simulink model "UAM_Hexa_PD_Obs_QGround"  (R2026a)
settings: Solver=ode4  StopTime=tf  FixedStep=0.01  EnableMultiTasking=on
values from neighbouring files (symbols this model uses):
  ArmConstants = struct('l1_dim', l1_dim,                        'l2_dim', l2_dim,                        'Hexa_to_joint_L', L,                        'Mass1', ml1,                        'Mass2', ml2,                        'Inertia1', Hl1,                        'Inertia2', Hl2,                        'MC1', c1,                        'MC2', c2,                        'Servos', Servos)    [init_model.m]    (also in init_var.m)
  HexaConstants = struct('Mass', mb,                         'Inertia', J ,                         'allo', allo,                          'invallo', invallo,                         'kT', kT)    [init_model.m]    (also in init_var.m)
  Observer = struct('E1', E1 ,     'E2', E2 ,     'E3', E3 ,     'E4', E4 ,     'MU1', MU1 ,     'MU2', MU2 ,     'MU3', MU3 ,     'alpha', alpha ,     'beta', beta)    [init_model.m]    (also in init_var.m)
libraries: px4Utilslib x189
(part 2 of 2)

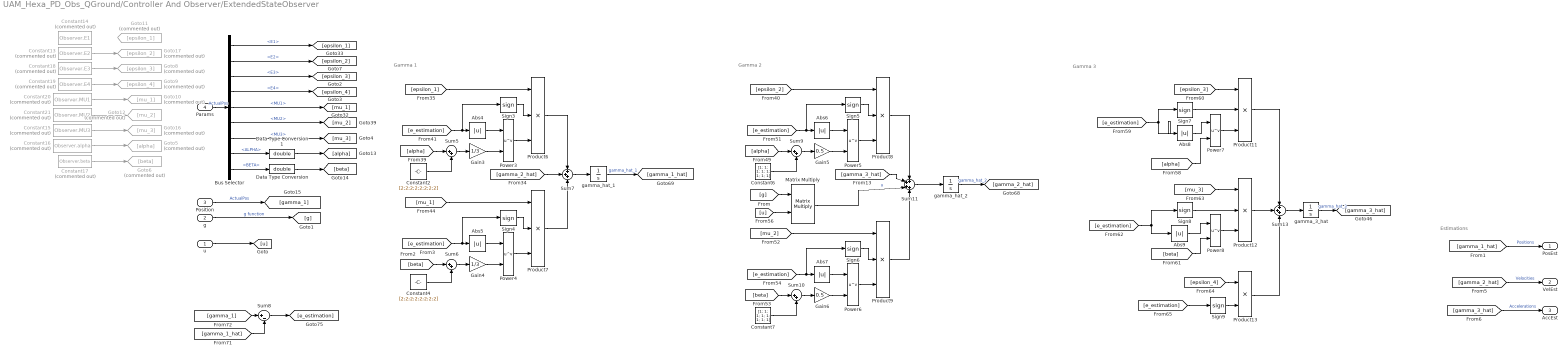
== system UAM_Hexa_PD_Obs_QGround/Controller And Observer/ExtendedStateObserver ==
  note: Estimations
  note: Gamma 3
  note: Gamma 2
  note: Gamma 1
  u : Inport  SampleTime=0.01
  g : Inport  Port=2  SampleTime=0.01
  Position : Inport  Port=3  SampleTime=0.01
  Params : Inport  Port=4  SampleTime=0.01
  Abs{4..9} (6 alike) : Abs  SaturateOnIntegerOverflow=off
  Bus Selector : BusSelector  OutputSignals=E1,E2,E3,E4,MU1,MU2,MU3,ALPHA,BETA
  Constant13 : Constant  Commented=on  Value=Observer.E2
  Constant14 : Constant  Commented=on  Value=Observer.E1
  Constant15 : Constant  Commented=on  Value=Observer.MU3
  Constant16 : Constant  Commented=on  Value=Observer.alpha
  Constant17 : Constant  Commented=on  Value=Observer.beta
  Constant18 : Constant  Commented=on  Value=Observer.E3
  Constant19 : Constant  Commented=on  Value=Observer.E4
  Constant2 : Constant  Value=[2;2;2;2;2;2;2;2]
  Constant20 : Constant  Commented=on  Value=Observer.MU1
  Constant21 : Constant  Commented=on  Value=Observer.MU2
  Constant4 : Constant  Value=[2;2;2;2;2;2;2;2]
  Constant6 : Constant  Value=[1; 1; 1; 1; 1; 1; 1; 1]
  Constant7 : Constant  Value=[1; 1; 1; 1; 1; 1; 1; 1]
  Data Type Conversion : DataTypeConversion  OutDataTypeStr=double  SaturateOnIntegerOverflow=off  RndMeth=Floor
  Data Type Conversion1 : DataTypeConversion  OutDataTypeStr=double  SaturateOnIntegerOverflow=off  RndMeth=Floor
  Gain3 : Gain  Gain=1/3
  Gain4 : Gain  Gain=1/3
  Gain5 : Gain  Gain=0.5
  Gain6 : Gain  Gain=0.5
  Goto10 : Goto  Commented=on  GotoTag=mu_1
  Goto11 : Goto  Commented=on  GotoTag=epsilon_1
  Goto12 : Goto  Commented=on  GotoTag=mu_2
  Goto16 : Goto  Commented=on  GotoTag=mu_3
  Goto17 : Goto  Commented=on  GotoTag=epsilon_2
  Goto5 : Goto  Commented=on  GotoTag=alpha
  Goto6 : Goto  Commented=on  GotoTag=beta
  Goto8 : Goto  Commented=on  GotoTag=epsilon_3
  Goto9 : Goto  Commented=on  GotoTag=epsilon_4
  Matrix Multiply : Product  Multiplication=Matrix(*)
  Power{3..8} (6 alike) : Math  Operator=pow
  Product{6..9,11..12} (6 alike) : Product  Inputs=3
  Product13 : Product
  Sign{3..9} (7 alike) : Signum
  Sum{5..6,9..10} (4 alike) : Sum  Inputs=|++
  Sum11 : Sum  Inputs=++++
  Sum13 : Sum  Inputs=+++
  Sum7 : Sum  Inputs=+++
  Sum8 : Sum  Inputs=|+-
  gamma_3_hat : Integrator  InitialCondition=[0; 0; -9.81; 0; 0; 0; 0; 0]
  gamma_hat_1 : Integrator  InitialCondition=[0; 0; 0.24; 0; 0; 0; 0; 0]
  gamma_hat_2 : Integrator  InitialCondition=zeros(8,1)
  PosEst : Outport  SampleTime=0.01
  VelEst : Outport  Port=2  SampleTime=0.01
  AccEst : Outport  Port=3  SampleTime=0.01
  wires:
  Bus Selector/8 -> Data Type Conversion1/1  "<ALPHA>"
  [beta] -> Sum10/1
  [e_estimation] -> Sign8/1, Abs9/1
  Power7/1 -> Product11/3
  Matrix Multiply/1 -> Sum11/3  "u"
  Bus Selector/9 -> Data Type Conversion/1  "<BETA>"
  [e_estimation] -> Abs8/1, Sign7/1
  [gamma_1_hat] -> PosEst/1  "Positions"
  Power8/1 -> Product12/3
  Constant4/1 -> Sum6/2
  [alpha] -> Sum5/1
  Product6/1 -> Sum7/1
  Abs8/1 -> Power7/1
  Power5/1 -> Product8/3
  [gamma_1] -> Sum8/1
  [e_estimation] -> Sign6/1, Abs7/1
  [epsilon_2] -> Product8/1
  Sum11/1 -> gamma_hat_2/1
  Bus Selector/7 -> [mu_3]  "<MU3>"
  Gain5/1 -> Power5/2
  [e_estimation] -> Sign3/1, Abs4/1
  Abs5/1 -> Power4/1
  Sum13/1 -> gamma_3_hat/1
  Abs7/1 -> Power6/1
  Product9/1 -> Sum11/4
  [epsilon_1] -> Product6/1
  Constant7/1 -> Sum10/2
  [epsilon_3] -> Product11/1
  Sum9/1 -> Gain5/1
  Sum6/1 -> Gain4/1
  [e_estimation] -> Sign5/1, Abs6/1
  u/1 -> [u]
  [mu_3] -> Product12/1
  Sign6/1 -> Product9/2
  Sum7/1 -> gamma_hat_1/1
  Sign8/1 -> Product12/2
  [alpha] -> Power7/2
  [epsilon_4] -> Product13/1
  [gamma_3_hat] -> Sum11/2
  [mu_1] -> Product7/1
  Sign3/1 -> Product6/2
  gamma_hat_2/1 -> [gamma_2_hat]  "gamma_hat_2"
  Bus Selector/2 -> [epsilon_2]  "<E2>"
  [mu_2] -> Product9/1
  Product11/1 -> Sum13/1
  [gamma_1_hat] -> Sum8/2
  Sign4/1 -> Product7/2
  Product7/1 -> Sum7/3
  Bus Selector/6 -> [mu_2]  "<MU2>"
  Bus Selector/1 -> [epsilon_1]  "<E1>"
  Constant6/1 -> Sum9/2
  Sign5/1 -> Product8/2
  [beta] -> Power8/2
  Constant2/1 -> Sum5/2
  Gain6/1 -> Power6/2
  Gain3/1 -> Power3/2
  Power6/1 -> Product9/3
  Position/1 -> [gamma_1]  "ActualPos"
  Bus Selector/4 -> [epsilon_4]  "<E4>"
  Product13/1 -> Sum13/3
  gamma_hat_1/1 -> [gamma_1_hat]  "gamma_hat_1"
  Sum5/1 -> Gain3/1
  Power3/1 -> Product6/3
  Power4/1 -> Product7/3
  Sum10/1 -> Gain6/1
  [gamma_2_hat] -> Sum7/2
  Sign7/1 -> Product11/2
  [beta] -> Sum6/1
  [e_estimation] -> Sign4/1, Abs5/1
  [e_estimation] -> Sign9/1
  Product8/1 -> Sum11/1
  Sign9/1 -> Product13/2
  Abs9/1 -> Power8/1
  [alpha] -> Sum9/1
  gamma_3_hat/1 -> [gamma_3_hat]  "gamma_hat_3"
  Sum8/1 -> [e_estimation]
  Gain4/1 -> Power4/2
  Bus Selector/5 -> [mu_1]  "<MU1>"
  Product12/1 -> Sum13/2
  g/1 -> [g]  "g function"
  Abs6/1 -> Power5/1
  Abs4/1 -> Power3/1
  [gamma_3_hat] -> AccEst/1  "Accelerations"
  [gamma_2_hat] -> VelEst/1  "Velocities"
  [g] -> Matrix Multiply/1
  [u] -> Matrix Multiply/2
  Params/1 -> Bus Selector/1  "ActualPos"
  Constant18/1 -> Goto8/1
  Constant20/1 -> Goto10/1
  Constant21/1 -> Goto12/1
  Constant15/1 -> Goto16/1
  Constant19/1 -> Goto9/1
  Constant17/1 -> Goto6/1
  Constant16/1 -> Goto5/1
  Constant13/1 -> Goto17/1
  Bus Selector/3 -> [epsilon_3]  "<E3>"
  Data Type Conversion/1 -> [beta]
  Data Type Conversion1/1 -> [alpha]

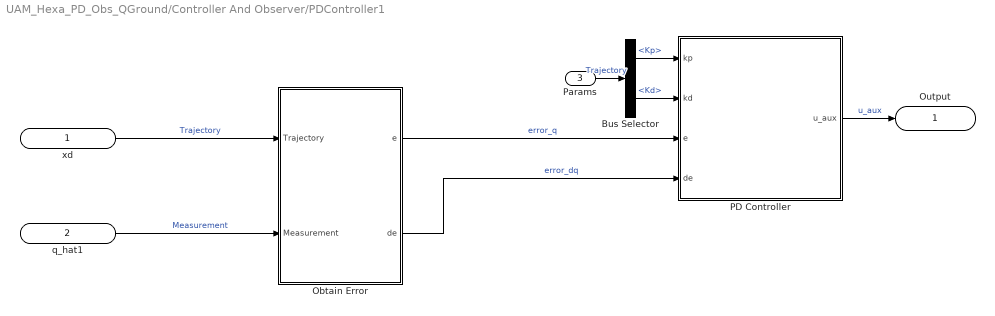
== system UAM_Hexa_PD_Obs_QGround/Controller And Observer/PDController1 ==
  xd : Inport
  q_hat1 : Inport  Port=2
  Params : Inport  Port=3
  Bus Selector : BusSelector  OutputSignals=Kp,Kd
  Obtain Error : Subsystem
  PD Controller : MATLAB Function  TreatAsAtomicUnit=on
  Output : Outport
  wires:
  xd/1 -> Obtain Error/1(Trajectory)  "Trajectory"
  q_hat1/1 -> Obtain Error/2(Measurement)  "Measurement"
  Obtain Error/1(e) -> PD Controller/3(e)  "error_q"
  Obtain Error/2(de) -> PD Controller/4(de)  "error_dq"
  Bus Selector/1 -> PD Controller/1(kp)  "<Kp>"
  Bus Selector/2 -> PD Controller/2(kd)  "<Kd>"
  PD Controller/1(u_aux) -> Output/1  "u_aux"
  Params/1 -> Bus Selector/1  "Trajectory"

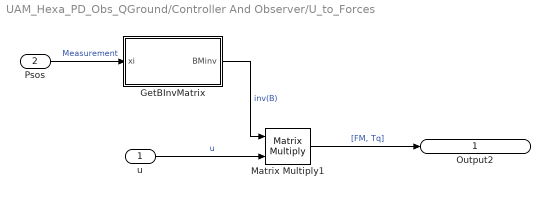
== system UAM_Hexa_PD_Obs_QGround/Controller And Observer/U_to_Forces ==
  u : Inport  SampleTime=0.01
  Psos : Inport  Port=2  SampleTime=0.01
  GetBInvMatrix : MATLAB Function  TreatAsAtomicUnit=on
  Matrix Multiply1 : Product  Multiplication=Matrix(*)
  Output2 : Outport  SampleTime=0.01
  wires:
  Psos/1 -> GetBInvMatrix/1(xi)  "Measurement"
  u/1 -> Matrix Multiply1/2  "u"
  Matrix Multiply1/1 -> Output2/1  "[FM, Tq]"
  GetBInvMatrix/1(BMinv) -> Matrix Multiply1/1  "inv(B)"

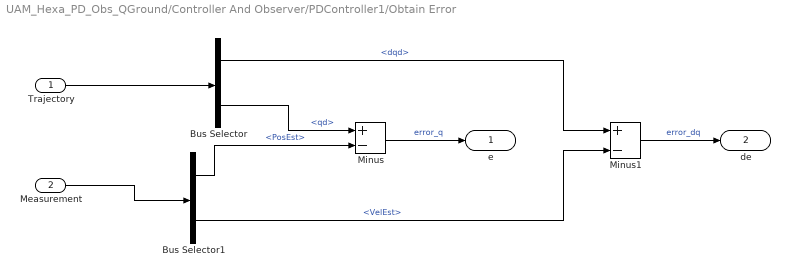
== system UAM_Hexa_PD_Obs_QGround/Controller And Observer/PDController1/Obtain Error ==
  Trajectory : Inport
  Measurement : Inport  Port=2
  Bus Selector : BusSelector  OutputSignals=dqd,qd
  Bus Selector1 : BusSelector  OutputSignals=PosEst,VelEst
  Minus : Sum  Inputs=+-
  Minus1 : Sum  Inputs=+-
  e : Outport
  de : Outport  Port=2
  wires:
  Bus Selector1/1 -> Minus/2  "<PosEst>"
  Bus Selector1/2 -> Minus1/2  "<VelEst>"
  Measurement/1 -> Bus Selector1/1
  Trajectory/1 -> Bus Selector/1
  Bus Selector/1 -> Minus1/1  "<dqd>"
  Bus Selector/2 -> Minus/1  "<qd>"
  Minus/1 -> e/1  "error_q"
  Minus1/1 -> de/1  "error_dq"

== matlab function UAM_Hexa_PD_Obs_QGround/Controller And Observer/PDController1/PD Controller ==
  data: kp input; kd input; u_aux output; e input; de input
function u_aux = pd_cont(kp, kd, e, de)


kp_m = [kp(1) 0       0     0     0       0     0     0;
        0     kp(2)   0     0     0       0     0     0;
        0     0       kp(3) 0     0       0     0     0;
        0     0       0     kp(4) 0       0     0     0;
        0     0       0     0     kp(5)   0     0     0;
        0     0       0     0     0       kp(6) 0     0;
        0     0       0     0     0       0     kp(7) 0;
        0     0       0     0     0       0     0     kp(8)];

kd_m = [kd(1) 0       0     0     0       0     0     0;
        0     kd(2)   0     0     0       0     0     0;
        0     0       kd(3) 0     0       0     0     0;
        0     0       0     kd(4) 0       0     0     0;
        0     0       0     0     kd(5)   0     0     0;
        0     0       0     0     0       kd(6) 0     0;
        0     0       0     0     0       0     kd(7) 0;
        0     0       0     0     0       0     0     kd(8)];


%v = ddP + kp_m * e + kd_m * de;
u_aux = kp_m * e + kd_m * de;
%v = ddP;

end

== matlab function UAM_Hexa_PD_Obs_QGround/Controller And Observer/MATLAB Function1 ==
  data: q input; dq input; HexaConstants parameter; ginv output; g output; fx output; ArmConstants parameter
function [ginv, g, fx] = Get_DCG_Hexa(q, dq, HexaConstants, ArmConstants)

DM = DMatrix(q, HexaConstants, ArmConstants);
CM = CMatrix(q, dq, HexaConstants, ArmConstants);
Gv = GVector(q, HexaConstants, ArmConstants);

g = inv(DM);
ginv = DM;

fx = DM\( -CM*dq - Gv );

end

== matlab function UAM_Hexa_PD_Obs_QGround/Controller And Observer/U_to_Forces/GetBInvMatrix ==
  data: xi input; BMinv output
function BMinv = GetBInvMatrix(xi)

% phi = xi(4);
% th  = xi(5);
% psi = xi(6);
% 
% BM1=[cos(phi)*cos(th),-cos(phi)*sin(psi)+cos(psi)*sin(phi)*sin(th), ...
%     sin(phi)*sin(psi)+cos(phi)*cos(psi)*sin(th),0,0,0;...
%     cos(th)*sin(psi), cos(phi)*cos(psi)+sin(phi)*sin(psi)*sin(th),...
%     -cos(psi)*sin(phi)+cos(phi)*sin(psi)*sin(phi),0,0,0;...
%     -sin(th),cos(th)*sin(psi),cos(phi)*cos(th),0,0,0;...
%     0,0,0,1,sin(phi)*tan(th),cos(phi)*tan(th);...
%     0,0,0,0,cos(phi),-sin(phi);0,0,0,0,sec(th)*sin(phi),cos(phi)*sec(th)];

BM1 = BMatrix(xi);

BM = blkdiag(BM1, eye(2,2));

BMinv = inv(BM);

end
